simulink model "zad2"  (R2025b)
settings: Solver=ode15s  StartTime=0.0  StopTime=1000  FixedStep=0.01  RelTol=1e-3
libraries: fuzblock x2
settings Model: LastModifiedBy=Anastasija

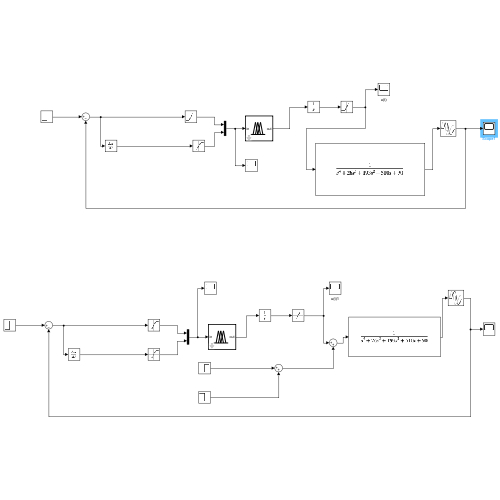
[thumbnail: Simulink's stored preview of the top-level diagram]
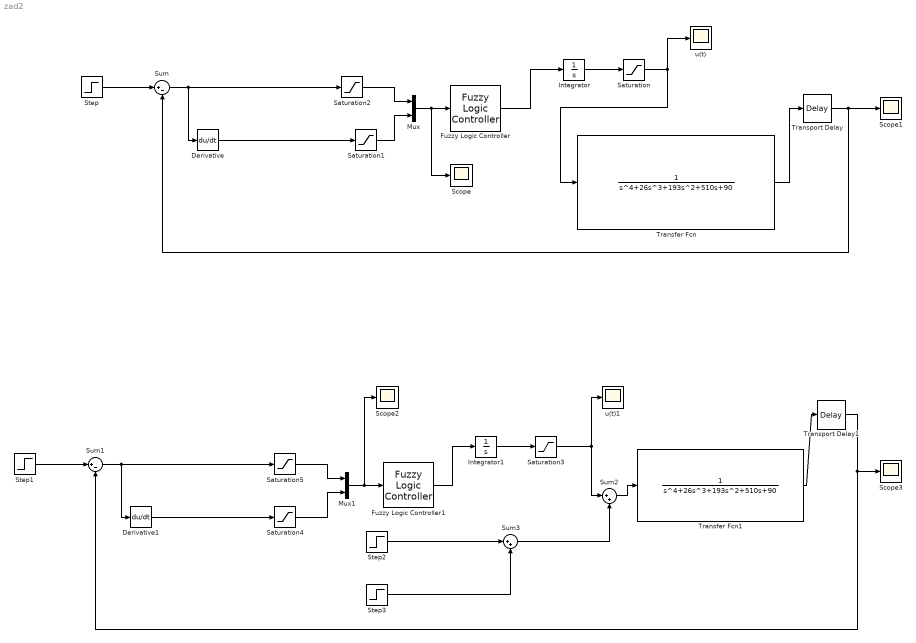
== system zad2 ==
  Derivative : Derivative
  Derivative1 : Derivative
  Fuzzy Logic Controller : fuzblock/Fuzzy Logic  Controller  FIS='fuzzyPI.fis'  OutputSampleNumber=101  DataType=double  UseLookupTable=off  NumBreakpoints=10  FuzzifiedInputs=off  RuleFiringStrengths=off  RuleOutputs=off  AggregatedOutputs=off  SimulateUsing=Interpreted execution  OutOfRangeInputValueMessage=warning  NoRuleFiredMessage=warning  EmptyOutputFuzzySetMessage=warning
  Fuzzy Logic Controller1 : fuzblock/Fuzzy Logic  Controller  FIS='fuzzyPI.fis'  OutputSampleNumber=101  DataType=double  UseLookupTable=off  NumBreakpoints=10  FuzzifiedInputs=off  RuleFiringStrengths=off  RuleOutputs=off  AggregatedOutputs=off  SimulateUsing=Interpreted execution  OutOfRangeInputValueMessage=warning  NoRuleFiredMessage=warning  EmptyOutputFuzzySetMessage=warning
  Integrator : Integrator
  Integrator1 : Integrator
  Mux : Mux  Inputs=2
  Mux1 : Mux  Inputs=2
  Saturation : Saturate  UpperLimit=100  LowerLimit=-100
  Saturation{1..2,4..5} (4 alike) : Saturate  UpperLimit=1  LowerLimit=-1
  Saturation3 : Saturate  UpperLimit=100  LowerLimit=-100
  Scope{,1..3} (4 alike) : Scope
      Scope settings: ActiveDisplayYMinimum=-0.575  ActiveDisplayYMaximum=1.175  DataLoggingVariableName=ScopeData2
      Scope1 settings: ActiveDisplayYMinimum=-2.224498912241418  ActiveDisplayYMaximum=2.1786300116410517
      Scope2 settings: ActiveDisplayYMinimum=-1.5300045960511235  ActiveDisplayYMaximum=1.7525639349991435  DataLoggingVariableName=ScopeData3
      Scope3 settings: ActiveDisplayYMinimum=-1.1363768367603071  ActiveDisplayYMaximum=0.65503665279547219  DataLoggingVariableName=ScopeData4
  Step : Step  Time=250  Before=-0.4  After=0.4  SampleTime=0
  Step1 : Step  Time=0  After=0  SampleTime=0
  Step2 : Step  Time=250  After=50  SampleTime=0
  Step3 : Step  Time=500  After=-100  SampleTime=0
  Sum : Sum  Inputs=|+-
  Sum1 : Sum  Inputs=|+-
  Sum2 : Sum  Inputs=|++
  Sum3 : Sum  Inputs=|++
  Transfer Fcn : TransferFcn  Denominator=[1 26 193 510 90]
  Transfer Fcn1 : TransferFcn  Denominator=[1 26 193 510 90]
  Transport Delay : TransportDelay  DelayTime=4
  Transport Delay1 : TransportDelay  DelayTime=4
  u(t) : Scope
      settings: ActiveDisplayYMinimum=-57.053640746889585  ActiveDisplayYMaximum=49.137333207589293
  u(t)1 : Scope
      settings: ActiveDisplayYMinimum=-63.876952793882538  ActiveDisplayYMaximum=30.588610788489767  DataLoggingVariableName=ScopeData5
  wires:
  Derivative/1 -> Saturation1/1
  Mux/1 -> Scope/1, Fuzzy Logic Controller/1
  Sum/1 -> Saturation2/1, Derivative/1
  Saturation1/1 -> Mux/2
  Integrator/1 -> Saturation/1
  Transfer Fcn/1 -> Transport Delay/1
  Transport Delay/1 -> Sum/2, Scope1/1
  Saturation/1 -> u(t)/1, Transfer Fcn/1
  Saturation2/1 -> Mux/1
  Fuzzy Logic Controller/1 -> Integrator/1
  Step/1 -> Sum/1
  Saturation5/1 -> Mux1/1
  Fuzzy Logic Controller1/1 -> Integrator1/1
  Transport Delay1/1 -> Sum1/2, Scope3/1
  Integrator1/1 -> Saturation3/1
  Transfer Fcn1/1 -> Transport Delay1/1
  Sum1/1 -> Saturation5/1, Derivative1/1
  Saturation3/1 -> Sum2/1, u(t)1/1
  Derivative1/1 -> Saturation4/1
  Mux1/1 -> Scope2/1, Fuzzy Logic Controller1/1
  Saturation4/1 -> Mux1/2
  Step1/1 -> Sum1/1
  Sum2/1 -> Transfer Fcn1/1
  Step2/1 -> Sum3/1
  Step3/1 -> Sum3/2
  Sum3/1 -> Sum2/2
